simulink model "gyro_3dof"  (R2025a)
settings: Solver=VariableStepAuto  StartTime=0.0  StopTime=10  RelTol=1e-3
libraries: simulink x5, rllib x1
settings Model: Creator=Sundar dell  LastModifiedBy=Mohan Aneesh

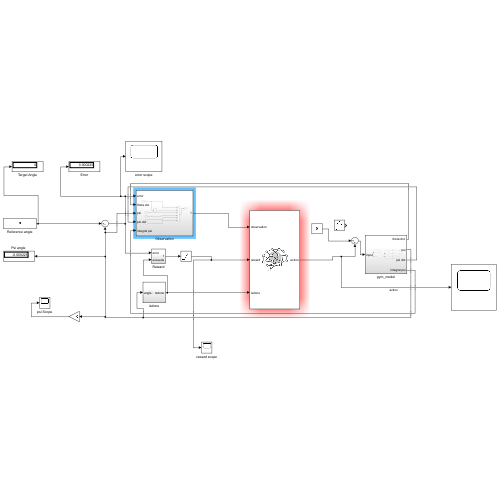
[thumbnail: Simulink's stored preview of the top-level diagram]
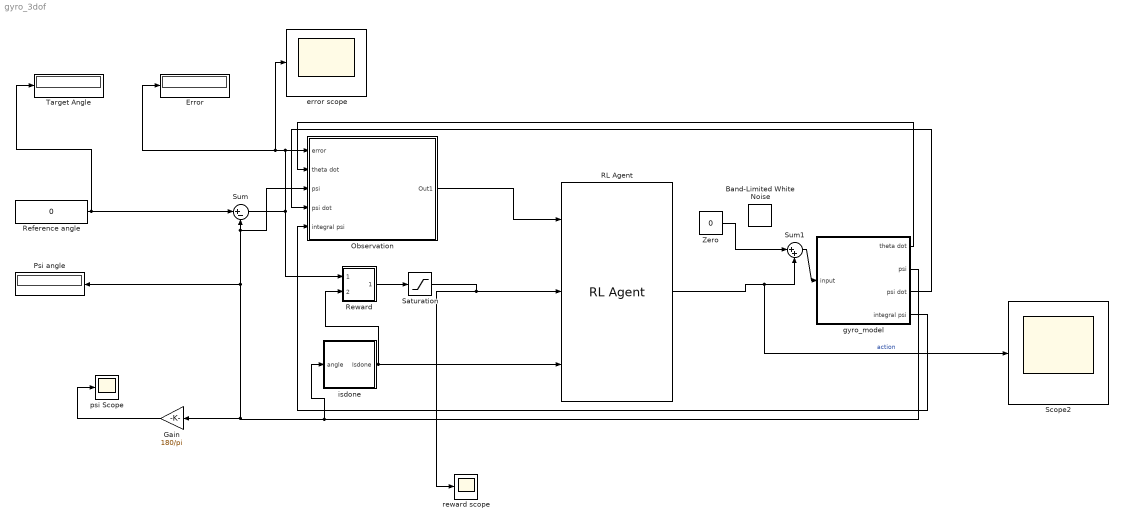
== system gyro_3dof ==
  Band-Limited White Noise : simulink/Sources/Band-Limited White Noise  Cov=[0.00001]  Ts=0.1  seed=[23341]
  Error : Display
  Gain : Gain  Gain=180/pi
  Observation : Subsystem
  "Psi angle " : Display
  RL Agent : rllib/RL Agent  Agent=agentObj  ExternalActionAsInput=off  ProvideLastAction=off  ProvideCumRwd=off  TreatAsDirectFeedthrough=on  UseStrictObservationDataTypes=off
  Reference angle : Constant  Value=0
  Reward : Subsystem
  Saturation : Saturate  UpperLimit=inf  LowerLimit=-100
  Scope2 : Scope
      settings: ActiveDisplayYMinimum=-3.5933108925819397  ActiveDisplayYMaximum=3.1734047532081604  DataLoggingVariableName=ScopeData3
  Sum : Sum  Inputs=|+-
  Sum1 : Sum  Inputs=|++
  Target Angle : Display
  Zero : Constant  Value=0  OutDataTypeStr=Inherit: Inherit via back propagation
  error scope : Scope
      settings: ActiveDisplayYMinimum=-0.016561208811370007  ActiveDisplayYMaximum=0.13758777604551875  DataLoggingVariableName=ScopeData5
  gyro_model : Subsystem
  isdone : Subsystem
  psi Scope : Scope
      settings: ActiveDisplayYMinimum=-54.062029475551888  ActiveDisplayYMaximum=106.00689216395021
  reward scope : Scope
      settings: ActiveDisplayYMinimum=-0.19804200192370039  ActiveDisplayYMaximum=1.1331157779915222  DataLoggingVariableName=ScopeData2
  wires:
  RL Agent/1 -> Sum1/2, Scope2/1  "action"
  isdone/1(Isdone) -> Reward/2(exceeds), RL Agent/3
  Observation/1(Out1) -> RL Agent/1
  Sum/1 -> error scope/1, Error/1, Observation/1(error), Reward/1(error)
  Reward/1(Out1) -> Saturation/1
  Reference angle/1 -> Target Angle/1, Sum/1
  gyro_model/2(psi) -> isdone/1(angle), Gain/1, Observation/3(psi), Sum/2, "Psi angle "/1
  gyro_model/1("theta dot ") -> Observation/2(theta dot)
  gyro_model/3(psi dot) -> Observation/4(psi dot)
  gyro_model/4(integral psi) -> Observation/5(integral psi)
  Saturation/1 -> reward scope/1, RL Agent/2
  Gain/1 -> psi Scope/1
  Sum1/1 -> gyro_model/1(input)
  Zero/1 -> Sum1/1

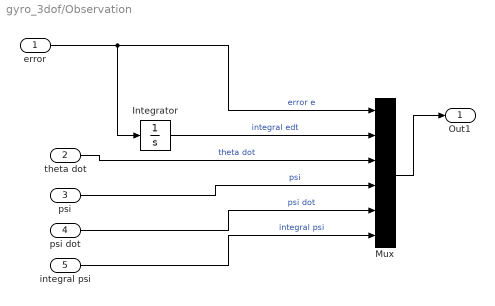
== system gyro_3dof/Observation ==
  error : Inport
  theta dot : Inport  Port=2
  psi : Inport  Port=3
  psi dot : Inport  Port=4
  integral psi : Inport  Port=5
  Integrator : Integrator
  Mux : Mux  Inputs=6
  Out1 : Outport
  wires:
  error/1 -> Integrator/1, Mux/1  "error e"
  Mux/1 -> Out1/1
  Integrator/1 -> Mux/2  "integral edt"
  theta dot/1 -> Mux/3  "theta dot"
  psi/1 -> Mux/4  "psi"
  psi dot/1 -> Mux/5  "psi dot"
  integral psi/1 -> Mux/6  "integral psi"

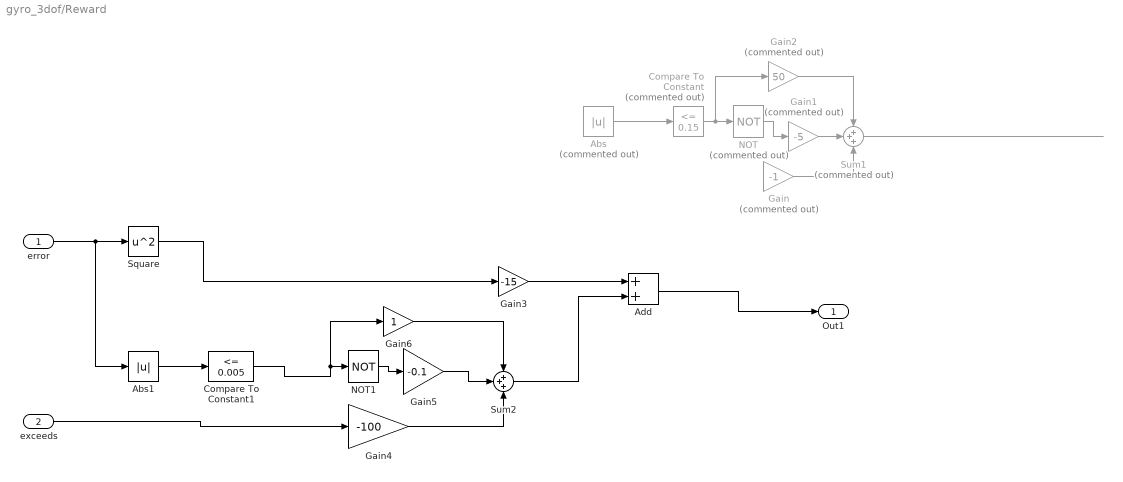
== system gyro_3dof/Reward ==
  error : Inport
  exceeds : Inport  Port=2
  Abs : Abs  Commented=on  SaturateOnIntegerOverflow=off
  Abs1 : Abs  SaturateOnIntegerOverflow=off
  Add : Sum
  Compare To Constant : simulink/Logic and Bit Operations/Compare To Constant  Commented=on  relop=<=  const=0.15  OutDataTypeStr=boolean
  Compare To Constant1 : simulink/Logic and Bit Operations/Compare To Constant  relop=<=  const=0.005  OutDataTypeStr=boolean
  Gain : Gain  Commented=on  Gain=-1
  Gain1 : Gain  Commented=on  Gain=-5
  Gain2 : Gain  Commented=on  Gain=50
  Gain3 : Gain  Gain=-15
  Gain4 : Gain  Gain=-100
  Gain5 : Gain  Gain=-0.1
  Gain6 : Gain
  NOT : Logic  Commented=on  Operator=NOT  IconShape=distinctive  AllPortsSameDT=off  OutDataTypeStr=boolean
  NOT1 : Logic  Operator=NOT  IconShape=distinctive  AllPortsSameDT=off  OutDataTypeStr=boolean
  Square : Math  Operator=square
  Sum1 : Sum  Commented=on  Inputs=+++
  Sum2 : Sum  Inputs=+++
  Out1 : Outport
  wires:
  Gain/1 -> Sum1/3
  ? -> Abs/1
  Gain1/1 -> Sum1/2
  Gain2/1 -> Sum1/1
  NOT/1 -> Gain1/1
  Compare To Constant/1 -> Gain2/1, NOT/1
  Sum1/1 -> ?
  Abs/1 -> Compare To Constant/1
  error/1 -> Abs1/1, Square/1
  Square/1 -> Gain3/1
  Gain3/1 -> Add/1
  Abs1/1 -> Compare To Constant1/1
  Compare To Constant1/1 -> NOT1/1, Gain6/1
  NOT1/1 -> Gain5/1
  Gain6/1 -> Sum2/1
  Gain5/1 -> Sum2/2
  exceeds/1 -> Gain4/1
  Gain4/1 -> Sum2/3
  Sum2/1 -> Add/2
  Add/1 -> Out1/1

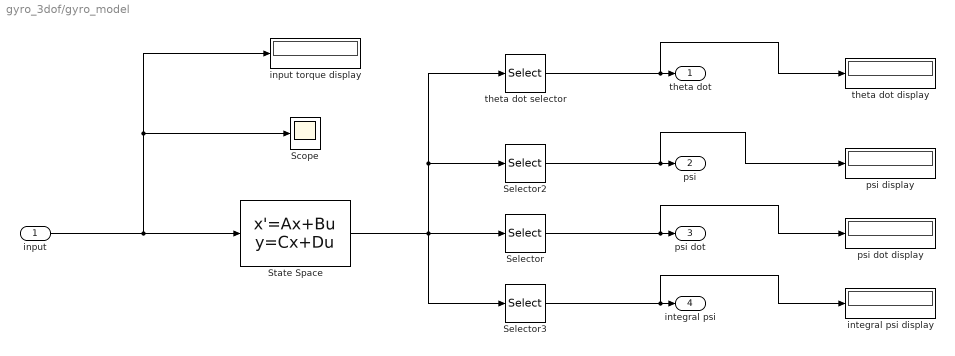
== system gyro_3dof/gyro_model ==
  input : Inport
  " input torque display" : Display
  Scope : Scope
      settings: ActiveDisplayYMinimum=-4.8353982418775558  ActiveDisplayYMaximum=1.554830476641655
  Selector : Selector  InputPortWidth=4  IndexOptions=Index vector (dialog)  Indices=[3]  OutputSizes=1
  Selector2 : Selector  InputPortWidth=4  IndexOptions=Index vector (dialog)  Indices=[2]  OutputSizes=1
  Selector3 : Selector  InputPortWidth=4  IndexOptions=Index vector (dialog)  Indices=[4]  OutputSizes=1
  State Space : StateSpace  A=[0 0 -112.8205 0; 0 0 1 0; 19.7309 0 0 0; 0 1 0 0]  B=[256.4102; 0; 0; 0]  C=diag([1,1,1,1])  D=zeros(4,1)  InitialCondition=[0;pi/2;0;0]
  integral psi display : Display
  psi display : Display
  psi dot display : Display
  theta dot display : Display
  theta dot selector : Selector  InputPortWidth=4  IndexOptions=Index vector (dialog)  Indices=[1]  OutputSizes=1
  "theta dot " : Outport
  psi : Outport  Port=2
  psi dot : Outport  Port=3
  integral psi : Outport  Port=4
  wires:
  input/1 -> " input torque display"/1, Scope/1, State Space/1
  theta dot selector/1 -> theta dot display/1, "theta dot "/1
  Selector2/1 -> psi display/1, psi/1
  Selector/1 -> psi dot display/1, psi dot/1
  Selector3/1 -> integral psi display/1, integral psi/1
  State Space/1 -> Selector/1, Selector2/1, theta dot selector/1, Selector3/1

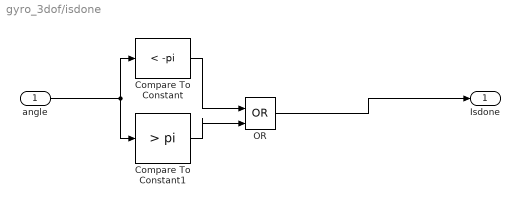
== system gyro_3dof/isdone ==
  angle : Inport
  Compare To Constant : simulink/Logic and Bit Operations/Compare To Constant  relop=<  const=-pi  OutDataTypeStr=boolean
  Compare To Constant1 : simulink/Logic and Bit Operations/Compare To Constant  relop=>  const=pi  OutDataTypeStr=boolean
  OR : Logic  Operator=OR  IconShape=distinctive  AllPortsSameDT=off  OutDataTypeStr=boolean
  Isdone : Outport
  wires:
  angle/1 -> Compare To Constant1/1, Compare To Constant/1
  Compare To Constant1/1 -> OR/2
  Compare To Constant/1 -> OR/1
  OR/1 -> Isdone/1
